simulink model "gm_HDLCrestFactorReduction"  (R2026a)
settings: Solver=FixedStepDiscrete  StopTime=stopTime
undefined symbols (not defined in the file or in its folder): ofdmSampleRate
libraries: dspsrcs4 x2, simulink x1
settings Model: Creator=The MathWorks, Inc.  LastModifiedBy=taokhe
settings OptimizationCC: ConditionallyExecuteInputs=off  InheritOutputTypeSmallerThanSingle=on
settings DebuggingCC: ArtificialAlgebraicLoopMsg=error  InheritedTsInSrcMsg=none  SingleTaskRateTransMsg=error
settings HardwareCC: ProdHWDeviceType=ASIC/FPGA->ASIC/FPGA  TargetBitPerLong=64.0  TargetBitPerPointer=64.0  TargetBitPerSizeT=64.0  TargetBitPerPtrDiffT=64.0  TargetLongLongMode=on  TargetIntDivRoundTo=Zero  TargetEndianess=LittleEndian  TargetWordSize=64.0  TargetHWDeviceType=Custom Processor->MATLAB Host Computer  ProdEqTarget=off

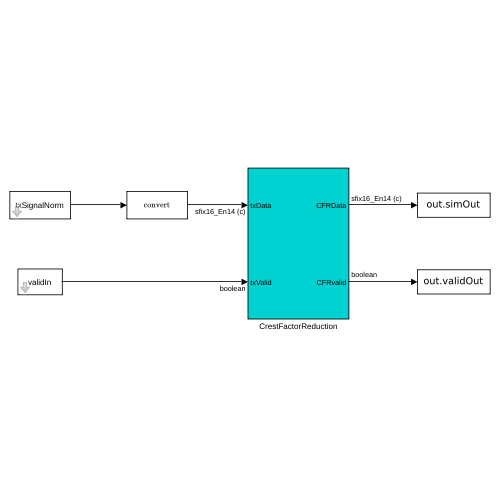
[thumbnail: Simulink's stored preview of the top-level diagram]
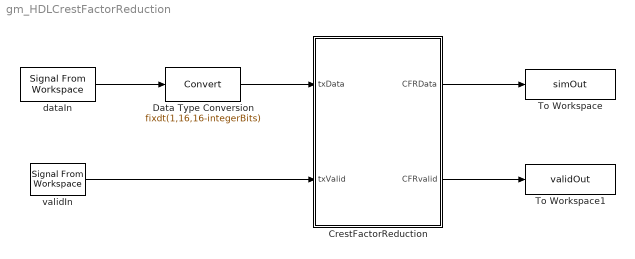
== system gm_HDLCrestFactorReduction ==
  CrestFactorReduction : Subsystem
  Data Type Conversion : DataTypeConversion  OutDataTypeStr=fixdt(1,16,16-integerBits)  SaturateOnIntegerOverflow=off  RndMeth=Floor
  To Workspace : ToWorkspace  VariableName=simOut  SampleTime=-1
      settings: Save2DSignal=2-D array (concatenate along first dimension)
  To Workspace1 : ToWorkspace  VariableName=validOut  SampleTime=-1
      settings: Save2DSignal=2-D array (concatenate along first dimension)
  dataIn : dspsrcs4/Signal From Workspace  X=txSignalNorm  Ts=1/ofdmSampleRate  nsamps=1  OutputAfterFinalValue=Setting to zero  ignoreOrWarnInputAndFrameLengths=off  OutputFrames=off
  validIn : dspsrcs4/Signal From Workspace  X=validIn  Ts=1/ofdmSampleRate  nsamps=1  OutputAfterFinalValue=Setting to zero  ignoreOrWarnInputAndFrameLengths=off  OutputFrames=off
  wires:
  validIn/1 -> CrestFactorReduction/2(txValid)
  Data Type Conversion/1 -> CrestFactorReduction/1(txData)
  CrestFactorReduction/2(CFRvalid) -> To Workspace1/1
  CrestFactorReduction/1(CFRData) -> To Workspace/1
  dataIn/1 -> Data Type Conversion/1

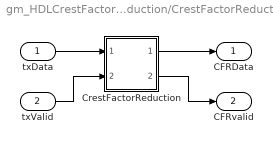
== system gm_HDLCrestFactorReduction/CrestFactorReduction ==
  txData : Inport  OutDataTypeStr=fixdt(1, 16, 14)  PortDimensions=1  SampleTime=5.20833333333333e-07
      settings: SignalType=complex
  txValid : Inport  Port=2  OutDataTypeStr=boolean  PortDimensions=1  SampleTime=5.20833333333333e-07
  CrestFactorReduction : Subsystem  mask{Threshold=0.7}
  CFRData : Outport  OutDataTypeStr=fixdt(1, 16, 14)  PortDimensions=1  SampleTime=5.20833333333333e-07
      settings: SignalType=complex
  CFRvalid : Outport  Port=2  OutDataTypeStr=boolean  PortDimensions=1  SampleTime=5.20833333333333e-07
  wires:
  CrestFactorReduction/2(CFRvalid) -> CFRvalid/1
  CrestFactorReduction/1(CFRData) -> CFRData/1
  txValid/1 -> CrestFactorReduction/2(valid)
  txData/1 -> CrestFactorReduction/1(data)

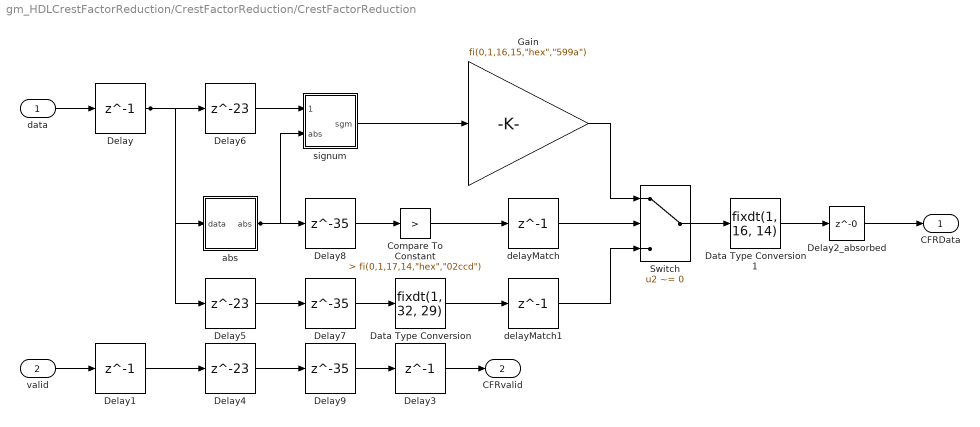
== system gm_HDLCrestFactorReduction/CrestFactorReduction/CrestFactorReduction ==
  data : Inport  OutDataTypeStr=fixdt(1, 16, 14)  PortDimensions=1  SampleTime=5.20833333333333e-07
      settings: SignalType=complex
  valid : Inport  Port=2  OutDataTypeStr=boolean  PortDimensions=1  SampleTime=5.20833333333333e-07
  Compare To Constant : simulink/Logic and Bit Operations/Compare To Constant  relop=>  const="fi(0,1,17,14,\"hex\",\"02ccd\")"  OutDataTypeStr=boolean
  Data Type Conversion : DataTypeConversion  OutDataTypeStr=fixdt(1, 32, 29)  SampleTime=5.20833333333333e-07  SaturateOnIntegerOverflow=off  RndMeth=Floor
  Data Type Conversion1 : DataTypeConversion  OutDataTypeStr=fixdt(1, 16, 14)  SampleTime=5.20833333333333e-07  SaturateOnIntegerOverflow=off  RndMeth=Floor
  Delay : Delay  DelayLength=1  InitialCondition=0  SampleTime=5.20833333333333e-07
  Delay1 : Delay  DelayLength=1  InitialCondition=0  SampleTime=5.20833333333333e-07
  Delay2_absorbed : Delay  DelayLength=0
  Delay3 : Delay  DelayLength=1  InitialCondition=0  SampleTime=5.20833333333333e-07
  Delay4 : Delay  DelayLength=23  InitialCondition=0  SampleTime=5.20833333333333e-07
  Delay5 : Delay  DelayLength=23  InitialCondition=0  SampleTime=5.20833333333333e-07
  Delay6 : Delay  DelayLength=23  InitialCondition=0  SampleTime=5.20833333333333e-07
  Delay7 : Delay  DelayLength=35  InitialCondition=0  SampleTime=5.20833333333333e-07
  Delay8 : Delay  DelayLength=35  InitialCondition=0  SampleTime=5.20833333333333e-07
  Delay9 : Delay  DelayLength=35  InitialCondition=0  SampleTime=5.20833333333333e-07
  Gain : Gain  Gain="fi(0,1,16,15,\"hex\",\"599a\")"  ParamDataTypeStr=fixdt(1, 16, 15)  OutDataTypeStr=fixdt(1, 32, 29)  SampleTime=5.20833333333333e-07
  Switch : Switch  Criteria=u2 ~= 0  Threshold="fi(0,0,1,0,\"hex\",\"0\")"  OutDataTypeStr=fixdt(1, 32, 29)  SampleTime=5.20833333333333e-07  SaturateOnIntegerOverflow=off  InputSameDT=off
  abs : Subsystem
  delayMatch : Delay  DelayLength=1  InitialCondition=0  SampleTime=5.20833333333333e-07
  delayMatch1 : Delay  DelayLength=1  InitialCondition=0  SampleTime=5.20833333333333e-07
  signum : Subsystem
  CFRData : Outport  OutDataTypeStr=fixdt(1, 16, 14)  PortDimensions=1  SampleTime=5.20833333333333e-07
      settings: SignalType=complex
  CFRvalid : Outport  Port=2  OutDataTypeStr=boolean  PortDimensions=1  SampleTime=5.20833333333333e-07
  wires:
  delayMatch1/1 -> Switch/3
  Delay3/1 -> CFRvalid/1
  Data Type Conversion/1 -> delayMatch1/1
  data/1 -> Delay/1
  valid/1 -> Delay1/1
  Delay6/1 -> signum/1(data)
  abs/1(abs) -> signum/2(abs), Delay8/1
  delayMatch/1 -> Switch/2
  Delay7/1 -> Data Type Conversion/1
  Delay2_absorbed/1 -> CFRData/1
  Delay1/1 -> Delay4/1
  Delay5/1 -> Delay7/1
  Delay4/1 -> Delay9/1
  Data Type Conversion1/1 -> Delay2_absorbed/1
  Gain/1 -> Switch/1
  signum/1(sgm) -> Gain/1
  Switch/1 -> Data Type Conversion1/1
  Delay8/1 -> Compare To Constant/1
  Delay9/1 -> Delay3/1
  Delay/1 -> abs/1(data), Delay5/1, Delay6/1
  Compare To Constant/1 -> delayMatch/1

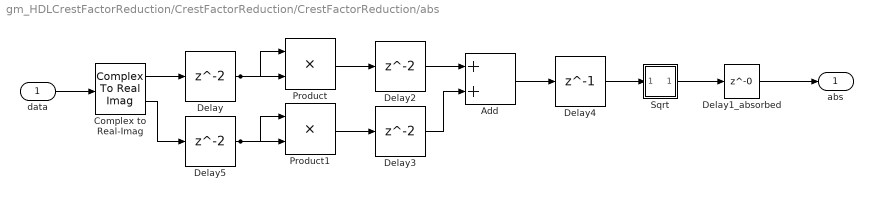
== system gm_HDLCrestFactorReduction/CrestFactorReduction/CrestFactorReduction/abs ==
  data : Inport  OutDataTypeStr=fixdt(1, 16, 14)  PortDimensions=1  SampleTime=5.20833333333333e-07
      settings: SignalType=complex
  Add : Sum  OutDataTypeStr=fixdt(1, 33, 28)  AccumDataTypeStr=fixdt(1, 33, 28)  SampleTime=5.20833333333333e-07
  Complex to Real-Imag : ComplexToRealImag  SampleTime=5.20833333333333e-07
  Delay{,2..3,5} (4 alike) : Delay  InitialCondition=0  SampleTime=5.20833333333333e-07
  Delay1_absorbed : Delay  DelayLength=0
  Delay4 : Delay  DelayLength=1  InitialCondition=0  SampleTime=5.20833333333333e-07
  Product : Product  Inputs=**  OutDataTypeStr=fixdt(1, 32, 28)  SampleTime=5.20833333333333e-07
  Product1 : Product  Inputs=**  OutDataTypeStr=fixdt(1, 32, 28)  SampleTime=5.20833333333333e-07
  Sqrt : Subsystem
  abs : Outport  OutDataTypeStr=fixdt(1, 17, 14)  PortDimensions=1  SampleTime=5.20833333333333e-07
  wires:
  Sqrt/1(Out1) -> Delay1_absorbed/1
  Delay4/1 -> Sqrt/1(In1)
  Add/1 -> Delay4/1
  Delay3/1 -> Add/2
  Delay2/1 -> Add/1
  Product1/1 -> Delay3/1
  Product/1 -> Delay2/1
  Delay5/1 -> Product1/1, Product1/2
  Delay/1 -> Product/1, Product/2
  Complex to Real-Imag/2 -> Delay5/1
  Delay1_absorbed/1 -> abs/1
  Complex to Real-Imag/1 -> Delay/1
  data/1 -> Complex to Real-Imag/1

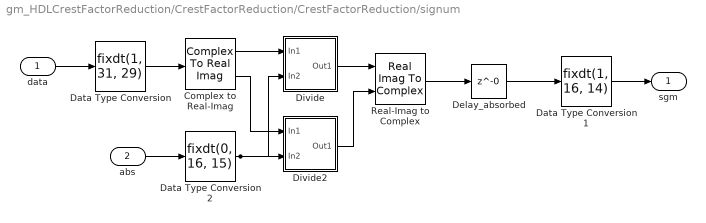
== system gm_HDLCrestFactorReduction/CrestFactorReduction/CrestFactorReduction/signum ==
  data : Inport  OutDataTypeStr=fixdt(1, 16, 14)  PortDimensions=1  SampleTime=5.20833333333333e-07
      settings: SignalType=complex
  abs : Inport  Port=2  OutDataTypeStr=fixdt(1, 17, 14)  PortDimensions=1  SampleTime=5.20833333333333e-07
  Complex to Real-Imag : ComplexToRealImag  SampleTime=5.20833333333333e-07
  Data Type Conversion : DataTypeConversion  OutDataTypeStr=fixdt(1, 31, 29)  SampleTime=5.20833333333333e-07  SaturateOnIntegerOverflow=off  RndMeth=Floor
  Data Type Conversion1 : DataTypeConversion  OutDataTypeStr=fixdt(1, 16, 14)  SampleTime=5.20833333333333e-07  SaturateOnIntegerOverflow=off  RndMeth=Floor
  Data Type Conversion2 : DataTypeConversion  OutDataTypeStr=fixdt(0, 16, 15)  SampleTime=5.20833333333333e-07  SaturateOnIntegerOverflow=off  RndMeth=Floor
  Delay_absorbed : Delay  DelayLength=0
  Divide : Subsystem
  Divide2 : Subsystem
  Real-Imag to Complex : RealImagToComplex  ConstantPart="fi(0,1,31,14,\"hex\",\"00000000\")"  SampleTime=5.20833333333333e-07
  sgm : Outport  OutDataTypeStr=fixdt(1, 16, 14)  PortDimensions=1  SampleTime=5.20833333333333e-07
      settings: SignalType=complex
  wires:
  Data Type Conversion1/1 -> sgm/1
  Delay_absorbed/1 -> Data Type Conversion1/1
  Divide/1(Out1) -> Real-Imag to Complex/1
  Real-Imag to Complex/1 -> Delay_absorbed/1
  Data Type Conversion2/1 -> Divide2/2(In2), Divide/2(In2)
  Complex to Real-Imag/2 -> Divide2/1(In1)
  Complex to Real-Imag/1 -> Divide/1(In1)
  abs/1 -> Data Type Conversion2/1
  Divide2/1(Out1) -> Real-Imag to Complex/2
  Data Type Conversion/1 -> Complex to Real-Imag/1
  data/1 -> Data Type Conversion/1

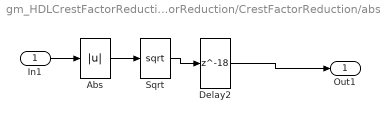
== system gm_HDLCrestFactorReduction/CrestFactorReduction/CrestFactorReduction/abs/Sqrt ==
  In1 : Inport
  Abs : Abs  RndMeth=Nearest
  Delay2 : Delay  DelayLength=18
  Sqrt : Sqrt  OutDataTypeStr=Inherit: Inherit via internal rule
  Out1 : Outport
  wires:
  In1/1 -> Abs/1
  Abs/1 -> Sqrt/1
  Sqrt/1 -> Delay2/1
  Delay2/1 -> Out1/1

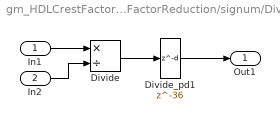
== system gm_HDLCrestFactorReduction/CrestFactorReduction/CrestFactorReduction/signum/Divide ==
  In1 : Inport
  In2 : Inport  Port=2
  Divide : Product  Inputs=*/  OutDataTypeStr=fixdt(1, 31, 14)  RndMeth=Zero  SaturateOnIntegerOverflow=on
  Divide_pd1 : Delay  DelayLength=36
  Out1 : Outport
  wires:
  Divide_pd1/1 -> Out1/1
  Divide/1 -> Divide_pd1/1
  In2/1 -> Divide/2
  In1/1 -> Divide/1

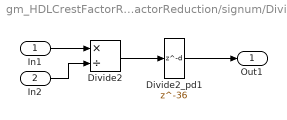
== system gm_HDLCrestFactorReduction/CrestFactorReduction/CrestFactorReduction/signum/Divide2 ==
  In1 : Inport
  In2 : Inport  Port=2
  Divide2 : Product  Inputs=*/  OutDataTypeStr=fixdt(1, 31, 14)  RndMeth=Zero  SaturateOnIntegerOverflow=on
  Divide2_pd1 : Delay  DelayLength=36
  Out1 : Outport
  wires:
  Divide2_pd1/1 -> Out1/1
  Divide2/1 -> Divide2_pd1/1
  In2/1 -> Divide2/2
  In1/1 -> Divide2/1
